simulink model "LOS_Tracking"  (R2021b)
settings: Solver=VariableStepAuto  StartTime=0.0  StopTime=273.72  RelTol=1e-3
values from neighbouring files (symbols this model uses):
  EL = out.EL    [plot_result.m]
undefined symbols (not defined in the file or in its folder): AZ, Optics
libraries: slpidlib x10, simulink_extras x10
(part 1 of 2)
settings Model: Creator=NGOC MAI  LastModifiedBy=NGOC MAI
settings DebuggingCC: UnconnectedInputMsg=none  UnconnectedOutputMsg=none  UnconnectedLineMsg=none
settings ModelReferenceCC: EnableRefExpFcnMdlSchedulingChecks=off
settings RTWCC: DLArmComputeVersion=20.02.1

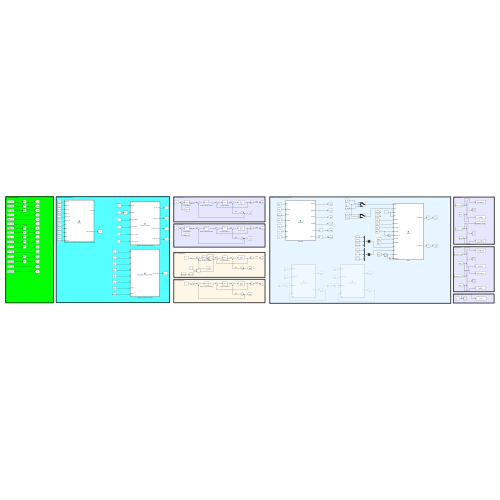
[thumbnail: Simulink's stored preview of the top-level diagram]
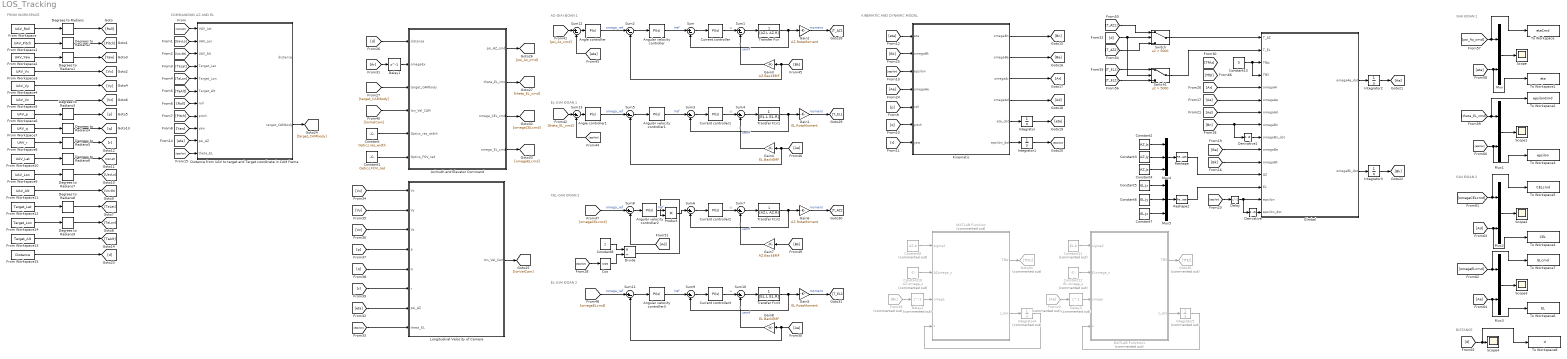
== system LOS_Tracking ==
  note: DISTANCE
  note: GIAI ĐOẠN 2
  note: GIAI ĐOẠN 1
  note: COMMANDING AZ AND EL
  note: FROM WORKSPACE
  note: KINEMATIC AND DYNAMIC MODEL
  note: AZ-GIAI ĐOẠN 1
  note: EL-GIAI ĐOẠN 1
  note: EL-GIAI ĐOẠN 2
  note: CEL-GIAI ĐOẠN 2
  Angle controller : slpidlib/PID Controller  Controller=P  Form=Parallel  TimeDomain=Continuous-time  UseExternalTs=off  SampleTime=-1  IntegratorMethod=Forward Euler  FilterMethod=Forward Euler  ControllerParametersSource=internal  P=AZ.KPpos  I=1  D=0  N=100  UseFilter=on  TunerSelectOption=Transfer Function Based (PID Tuner App)  InitialConditionSource=internal  InitialConditionForIntegrator=0  InitialConditionForFilter=0  DifferentiatorICPrevScaledInput=0  ExternalReset=none  TrackingMode=off  Kt=1  LimitOutput=off  SatLimitsSource=internal  UpperSaturationLimit=inf  LowerSaturationLimit=-inf  LinearizeAsGain=on  AntiWindupMode=none  Kb=1  POutMin=[]  POutMax=[]  IOutMin=[]  IOutMax=[]  DOutMin=[]  DOutMax=[]  NOutMin=[]  NOutMax=[]  SumOutMin=[]  SumOutMax=[]  SaturationOutMin=[]  SaturationOutMax=[]  PParamMin=[]  PParamMax=[]  IParamMin=[]  IParamMax=[]  DParamMin=[]  DParamMax=[]  NParamMin=[]  NParamMax=[]  KbParamMin=[]  KbParamMax=[]  KtParamMin=[]  KtParamMax=[]  KbOutMin=[]  KbOutMax=[]  KtOutMin=[]  KtOutMax=[]  IntegratorOutMin=[]  IntegratorOutMax=[]  FilterOutMin=[]  FilterOutMax=[]  SumI1OutMin=[]  SumI1OutMax=[]  SumI2OutMin=[]  SumI2OutMax=[]  SumI3OutMin=[]  SumI3OutMax=[]  SumI4OutMin=[]  SumI4OutMax=[]  SumDOutMin=[]  SumDOutMax=[]  DifferentiatorOutMin=[]  DifferentiatorOutMax=[]  FilterDiffOutCoefMin=[]  FilterDiffOutCoefMax=[]  ReciprocalOutMin=[]  ReciprocalOutMax=[]  SumDenOutMin=[]  SumDenOutMax=[]  SumNumOutMin=[]  SumNumOutMax=[]  DivideOutMin=[]  DivideOutMax=[]  UdiffTsProdOutMin=[]  UdiffTsProdOutMax=[]  NTsProdOutMin=[]  NTsProdOutMax=[]  UintegralTsProdOutMin=[]  UintegralTsProdOutMax=[]  UngainTsProdOutMin=[]  UngainTsProdOutMax=[]  IntegratorContinuousStateAttributes=''  IntegratorStateMustResolveToSignalObject=off  IntegratorRTWStateStorageClass=Auto  FilterContinuousStateAttributes=''  FilterStateMustResolveToSignalObject=off  FilterRTWStateStorageClass=Auto  ParallelPVariant=InternalParameters  IdealPVariant=Disabled  IVariant=Disabled  DVariant=Disabled  IntegratorVariant=Disabled  SatVariant=Disabled  AWVariant=Disabled  PCopyVariant=Disabled  TRVariant=Disabled  FdbkBlocksVariant=Forward  IdealPFdbkVariant=Disabled  SatFdbkVariant=Disabled  DerivativeFilterVariant=Disabled  NVariant=Disabled  NCopyVariant=Disabled_SignalSpec  FilterICVariant=Disabled  IntegratorICVariant=Disabled  ExternalResetVariant=Disabled  TRSumVariant=Passthrough  SumFdbkVariant=Disabled  SumVariant=Passthrough_P  TsampFilterVariant=InternalTs  TsampNgainVariant=Passthrough  TsampIntegralVariant=Disabled_SignalSpec  ExternalSaturationOutDataTypeStr=Inherit: Same as second input
  Angle controller1 : slpidlib/PID Controller  Controller=P  Form=Parallel  TimeDomain=Continuous-time  UseExternalTs=off  SampleTime=-1  IntegratorMethod=Forward Euler  FilterMethod=Forward Euler  ControllerParametersSource=internal  P=EL.KPpos  I=1  D=0  N=100  UseFilter=on  TunerSelectOption=Transfer Function Based (PID Tuner App)  InitialConditionSource=internal  InitialConditionForIntegrator=0  InitialConditionForFilter=0  DifferentiatorICPrevScaledInput=0  ExternalReset=none  TrackingMode=off  Kt=1  LimitOutput=off  SatLimitsSource=internal  UpperSaturationLimit=inf  LowerSaturationLimit=-inf  LinearizeAsGain=on  AntiWindupMode=none  Kb=1  POutMin=[]  POutMax=[]  IOutMin=[]  IOutMax=[]  DOutMin=[]  DOutMax=[]  NOutMin=[]  NOutMax=[]  SumOutMin=[]  SumOutMax=[]  SaturationOutMin=[]  SaturationOutMax=[]  PParamMin=[]  PParamMax=[]  IParamMin=[]  IParamMax=[]  DParamMin=[]  DParamMax=[]  NParamMin=[]  NParamMax=[]  KbParamMin=[]  KbParamMax=[]  KtParamMin=[]  KtParamMax=[]  KbOutMin=[]  KbOutMax=[]  KtOutMin=[]  KtOutMax=[]  IntegratorOutMin=[]  IntegratorOutMax=[]  FilterOutMin=[]  FilterOutMax=[]  SumI1OutMin=[]  SumI1OutMax=[]  SumI2OutMin=[]  SumI2OutMax=[]  SumI3OutMin=[]  SumI3OutMax=[]  SumI4OutMin=[]  SumI4OutMax=[]  SumDOutMin=[]  SumDOutMax=[]  DifferentiatorOutMin=[]  DifferentiatorOutMax=[]  FilterDiffOutCoefMin=[]  FilterDiffOutCoefMax=[]  ReciprocalOutMin=[]  ReciprocalOutMax=[]  SumDenOutMin=[]  SumDenOutMax=[]  SumNumOutMin=[]  SumNumOutMax=[]  DivideOutMin=[]  DivideOutMax=[]  UdiffTsProdOutMin=[]  UdiffTsProdOutMax=[]  NTsProdOutMin=[]  NTsProdOutMax=[]  UintegralTsProdOutMin=[]  UintegralTsProdOutMax=[]  UngainTsProdOutMin=[]  UngainTsProdOutMax=[]  IntegratorContinuousStateAttributes=''  IntegratorStateMustResolveToSignalObject=off  IntegratorRTWStateStorageClass=Auto  FilterContinuousStateAttributes=''  FilterStateMustResolveToSignalObject=off  FilterRTWStateStorageClass=Auto  ParallelPVariant=InternalParameters  IdealPVariant=Disabled  IVariant=Disabled  DVariant=Disabled  IntegratorVariant=Disabled  SatVariant=Disabled  AWVariant=Disabled  PCopyVariant=Disabled  TRVariant=Disabled  FdbkBlocksVariant=Forward  IdealPFdbkVariant=Disabled  SatFdbkVariant=Disabled  DerivativeFilterVariant=Disabled  NVariant=Disabled  NCopyVariant=Disabled_SignalSpec  FilterICVariant=Disabled  IntegratorICVariant=Disabled  ExternalResetVariant=Disabled  TRSumVariant=Passthrough  SumFdbkVariant=Disabled  SumVariant=Passthrough_P  TsampFilterVariant=InternalTs  TsampNgainVariant=Passthrough  TsampIntegralVariant=Disabled_SignalSpec  ExternalSaturationOutDataTypeStr=Inherit: Same as second input
  Angular velocity controller : slpidlib/PID Controller  Controller=PI  Form=Parallel  TimeDomain=Continuous-time  UseExternalTs=off  SampleTime=-1  IntegratorMethod=Forward Euler  FilterMethod=Forward Euler  ControllerParametersSource=internal  P=AZ.KPvel  I=AZ.KIvel  D=0  N=100  UseFilter=on  TunerSelectOption=Transfer Function Based (PID Tuner App)  InitialConditionSource=internal  InitialConditionForIntegrator=0  InitialConditionForFilter=0  DifferentiatorICPrevScaledInput=0  ExternalReset=none  TrackingMode=off  Kt=1  LimitOutput=off  SatLimitsSource=internal  UpperSaturationLimit=inf  LowerSaturationLimit=-inf  LinearizeAsGain=on  AntiWindupMode=none  Kb=1  POutMin=[]  POutMax=[]  IOutMin=[]  IOutMax=[]  DOutMin=[]  DOutMax=[]  NOutMin=[]  NOutMax=[]  SumOutMin=[]  SumOutMax=[]  SaturationOutMin=[]  SaturationOutMax=[]  PParamMin=[]  PParamMax=[]  IParamMin=[]  IParamMax=[]  DParamMin=[]  DParamMax=[]  NParamMin=[]  NParamMax=[]  KbParamMin=[]  KbParamMax=[]  KtParamMin=[]  KtParamMax=[]  KbOutMin=[]  KbOutMax=[]  KtOutMin=[]  KtOutMax=[]  IntegratorOutMin=[]  IntegratorOutMax=[]  FilterOutMin=[]  FilterOutMax=[]  SumI1OutMin=[]  SumI1OutMax=[]  SumI2OutMin=[]  SumI2OutMax=[]  SumI3OutMin=[]  SumI3OutMax=[]  SumI4OutMin=[]  SumI4OutMax=[]  SumDOutMin=[]  SumDOutMax=[]  DifferentiatorOutMin=[]  DifferentiatorOutMax=[]  FilterDiffOutCoefMin=[]  FilterDiffOutCoefMax=[]  ReciprocalOutMin=[]  ReciprocalOutMax=[]  SumDenOutMin=[]  SumDenOutMax=[]  SumNumOutMin=[]  SumNumOutMax=[]  DivideOutMin=[]  DivideOutMax=[]  UdiffTsProdOutMin=[]  UdiffTsProdOutMax=[]  NTsProdOutMin=[]  NTsProdOutMax=[]  UintegralTsProdOutMin=[]  UintegralTsProdOutMax=[]  UngainTsProdOutMin=[]  UngainTsProdOutMax=[]  IntegratorContinuousStateAttributes=''  IntegratorStateMustResolveToSignalObject=off  IntegratorRTWStateStorageClass=Auto  FilterContinuousStateAttributes=''  FilterStateMustResolveToSignalObject=off  FilterRTWStateStorageClass=Auto  ParallelPVariant=InternalParameters  IdealPVariant=Disabled  IVariant=InternalParameters  DVariant=Disabled  IntegratorVariant=Continuous  SatVariant=Disabled  AWVariant=Passthrough  PCopyVariant=Disabled  TRVariant=Disabled  FdbkBlocksVariant=Forward  IdealPFdbkVariant=Disabled  SatFdbkVariant=Disabled  DerivativeFilterVariant=Disabled  NVariant=Disabled  NCopyVariant=Disabled_SignalSpec  FilterICVariant=Disabled  IntegratorICVariant=InternalICs  ExternalResetVariant=Disabled  TRSumVariant=Passthrough  SumFdbkVariant=Disabled  SumVariant=Sum_PI  TsampFilterVariant=InternalTs  TsampNgainVariant=Passthrough  TsampIntegralVariant=Disabled_SignalSpec  ExternalSaturationOutDataTypeStr=Inherit: Same as second input
  Angular velocity controller1 : slpidlib/PID Controller  Controller=PI  Form=Parallel  TimeDomain=Continuous-time  UseExternalTs=off  SampleTime=-1  IntegratorMethod=Forward Euler  FilterMethod=Forward Euler  ControllerParametersSource=internal  P=EL.KPvel  I=EL.KIvel  D=0  N=100  UseFilter=on  TunerSelectOption=Transfer Function Based (PID Tuner App)  InitialConditionSource=internal  InitialConditionForIntegrator=0  InitialConditionForFilter=0  DifferentiatorICPrevScaledInput=0  ExternalReset=none  TrackingMode=off  Kt=1  LimitOutput=off  SatLimitsSource=internal  UpperSaturationLimit=inf  LowerSaturationLimit=-inf  LinearizeAsGain=on  AntiWindupMode=none  Kb=1  POutMin=[]  POutMax=[]  IOutMin=[]  IOutMax=[]  DOutMin=[]  DOutMax=[]  NOutMin=[]  NOutMax=[]  SumOutMin=[]  SumOutMax=[]  SaturationOutMin=[]  SaturationOutMax=[]  PParamMin=[]  PParamMax=[]  IParamMin=[]  IParamMax=[]  DParamMin=[]  DParamMax=[]  NParamMin=[]  NParamMax=[]  KbParamMin=[]  KbParamMax=[]  KtParamMin=[]  KtParamMax=[]  KbOutMin=[]  KbOutMax=[]  KtOutMin=[]  KtOutMax=[]  IntegratorOutMin=[]  IntegratorOutMax=[]  FilterOutMin=[]  FilterOutMax=[]  SumI1OutMin=[]  SumI1OutMax=[]  SumI2OutMin=[]  SumI2OutMax=[]  SumI3OutMin=[]  SumI3OutMax=[]  SumI4OutMin=[]  SumI4OutMax=[]  SumDOutMin=[]  SumDOutMax=[]  DifferentiatorOutMin=[]  DifferentiatorOutMax=[]  FilterDiffOutCoefMin=[]  FilterDiffOutCoefMax=[]  ReciprocalOutMin=[]  ReciprocalOutMax=[]  SumDenOutMin=[]  SumDenOutMax=[]  SumNumOutMin=[]  SumNumOutMax=[]  DivideOutMin=[]  DivideOutMax=[]  UdiffTsProdOutMin=[]  UdiffTsProdOutMax=[]  NTsProdOutMin=[]  NTsProdOutMax=[]  UintegralTsProdOutMin=[]  UintegralTsProdOutMax=[]  UngainTsProdOutMin=[]  UngainTsProdOutMax=[]  IntegratorContinuousStateAttributes=''  IntegratorStateMustResolveToSignalObject=off  IntegratorRTWStateStorageClass=Auto  FilterContinuousStateAttributes=''  FilterStateMustResolveToSignalObject=off  FilterRTWStateStorageClass=Auto  ParallelPVariant=InternalParameters  IdealPVariant=Disabled  IVariant=InternalParameters  DVariant=Disabled  IntegratorVariant=Continuous  SatVariant=Disabled  AWVariant=Passthrough  PCopyVariant=Disabled  TRVariant=Disabled  FdbkBlocksVariant=Forward  IdealPFdbkVariant=Disabled  SatFdbkVariant=Disabled  DerivativeFilterVariant=Disabled  NVariant=Disabled  NCopyVariant=Disabled_SignalSpec  FilterICVariant=Disabled  IntegratorICVariant=InternalICs  ExternalResetVariant=Disabled  TRSumVariant=Passthrough  SumFdbkVariant=Disabled  SumVariant=Sum_PI  TsampFilterVariant=InternalTs  TsampNgainVariant=Passthrough  TsampIntegralVariant=Disabled_SignalSpec  ExternalSaturationOutDataTypeStr=Inherit: Same as second input
  Angular velocity controller2 : slpidlib/PID Controller  Controller=PI  Form=Parallel  TimeDomain=Continuous-time  UseExternalTs=off  SampleTime=-1  IntegratorMethod=Forward Euler  FilterMethod=Forward Euler  ControllerParametersSource=internal  P=AZ.KPvel  I=AZ.KIvel  D=0  N=100  UseFilter=on  TunerSelectOption=Transfer Function Based (PID Tuner App)  InitialConditionSource=internal  InitialConditionForIntegrator=0  InitialConditionForFilter=0  DifferentiatorICPrevScaledInput=0  ExternalReset=none  TrackingMode=off  Kt=1  LimitOutput=off  SatLimitsSource=internal  UpperSaturationLimit=inf  LowerSaturationLimit=-inf  LinearizeAsGain=on  AntiWindupMode=none  Kb=1  POutMin=[]  POutMax=[]  IOutMin=[]  IOutMax=[]  DOutMin=[]  DOutMax=[]  NOutMin=[]  NOutMax=[]  SumOutMin=[]  SumOutMax=[]  SaturationOutMin=[]  SaturationOutMax=[]  PParamMin=[]  PParamMax=[]  IParamMin=[]  IParamMax=[]  DParamMin=[]  DParamMax=[]  NParamMin=[]  NParamMax=[]  KbParamMin=[]  KbParamMax=[]  KtParamMin=[]  KtParamMax=[]  KbOutMin=[]  KbOutMax=[]  KtOutMin=[]  KtOutMax=[]  IntegratorOutMin=[]  IntegratorOutMax=[]  FilterOutMin=[]  FilterOutMax=[]  SumI1OutMin=[]  SumI1OutMax=[]  SumI2OutMin=[]  SumI2OutMax=[]  SumI3OutMin=[]  SumI3OutMax=[]  SumI4OutMin=[]  SumI4OutMax=[]  SumDOutMin=[]  SumDOutMax=[]  DifferentiatorOutMin=[]  DifferentiatorOutMax=[]  FilterDiffOutCoefMin=[]  FilterDiffOutCoefMax=[]  ReciprocalOutMin=[]  ReciprocalOutMax=[]  SumDenOutMin=[]  SumDenOutMax=[]  SumNumOutMin=[]  SumNumOutMax=[]  DivideOutMin=[]  DivideOutMax=[]  UdiffTsProdOutMin=[]  UdiffTsProdOutMax=[]  NTsProdOutMin=[]  NTsProdOutMax=[]  UintegralTsProdOutMin=[]  UintegralTsProdOutMax=[]  UngainTsProdOutMin=[]  UngainTsProdOutMax=[]  IntegratorContinuousStateAttributes=''  IntegratorStateMustResolveToSignalObject=off  IntegratorRTWStateStorageClass=Auto  FilterContinuousStateAttributes=''  FilterStateMustResolveToSignalObject=off  FilterRTWStateStorageClass=Auto  ParallelPVariant=InternalParameters  IdealPVariant=Disabled  IVariant=InternalParameters  DVariant=Disabled  IntegratorVariant=Continuous  SatVariant=Disabled  AWVariant=Passthrough  PCopyVariant=Disabled  TRVariant=Disabled  FdbkBlocksVariant=Forward  IdealPFdbkVariant=Disabled  SatFdbkVariant=Disabled  DerivativeFilterVariant=Disabled  NVariant=Disabled  NCopyVariant=Disabled_SignalSpec  FilterICVariant=Disabled  IntegratorICVariant=InternalICs  ExternalResetVariant=Disabled  TRSumVariant=Passthrough  SumFdbkVariant=Disabled  SumVariant=Sum_PI  TsampFilterVariant=InternalTs  TsampNgainVariant=Passthrough  TsampIntegralVariant=Disabled_SignalSpec  ExternalSaturationOutDataTypeStr=Inherit: Same as second input
  Angular velocity controller3 : slpidlib/PID Controller  Controller=PI  Form=Parallel  TimeDomain=Continuous-time  UseExternalTs=off  SampleTime=-1  IntegratorMethod=Forward Euler  FilterMethod=Forward Euler  ControllerParametersSource=internal  P=EL.KPvel  I=EL.KIvel  D=0  N=100  UseFilter=on  TunerSelectOption=Transfer Function Based (PID Tuner App)  InitialConditionSource=internal  InitialConditionForIntegrator=0  InitialConditionForFilter=0  DifferentiatorICPrevScaledInput=0  ExternalReset=none  TrackingMode=off  Kt=1  LimitOutput=off  SatLimitsSource=internal  UpperSaturationLimit=inf  LowerSaturationLimit=-inf  LinearizeAsGain=on  AntiWindupMode=none  Kb=1  POutMin=[]  POutMax=[]  IOutMin=[]  IOutMax=[]  DOutMin=[]  DOutMax=[]  NOutMin=[]  NOutMax=[]  SumOutMin=[]  SumOutMax=[]  SaturationOutMin=[]  SaturationOutMax=[]  PParamMin=[]  PParamMax=[]  IParamMin=[]  IParamMax=[]  DParamMin=[]  DParamMax=[]  NParamMin=[]  NParamMax=[]  KbParamMin=[]  KbParamMax=[]  KtParamMin=[]  KtParamMax=[]  KbOutMin=[]  KbOutMax=[]  KtOutMin=[]  KtOutMax=[]  IntegratorOutMin=[]  IntegratorOutMax=[]  FilterOutMin=[]  FilterOutMax=[]  SumI1OutMin=[]  SumI1OutMax=[]  SumI2OutMin=[]  SumI2OutMax=[]  SumI3OutMin=[]  SumI3OutMax=[]  SumI4OutMin=[]  SumI4OutMax=[]  SumDOutMin=[]  SumDOutMax=[]  DifferentiatorOutMin=[]  DifferentiatorOutMax=[]  FilterDiffOutCoefMin=[]  FilterDiffOutCoefMax=[]  ReciprocalOutMin=[]  ReciprocalOutMax=[]  SumDenOutMin=[]  SumDenOutMax=[]  SumNumOutMin=[]  SumNumOutMax=[]  DivideOutMin=[]  DivideOutMax=[]  UdiffTsProdOutMin=[]  UdiffTsProdOutMax=[]  NTsProdOutMin=[]  NTsProdOutMax=[]  UintegralTsProdOutMin=[]  UintegralTsProdOutMax=[]  UngainTsProdOutMin=[]  UngainTsProdOutMax=[]  IntegratorContinuousStateAttributes=''  IntegratorStateMustResolveToSignalObject=off  IntegratorRTWStateStorageClass=Auto  FilterContinuousStateAttributes=''  FilterStateMustResolveToSignalObject=off  FilterRTWStateStorageClass=Auto  ParallelPVariant=InternalParameters  IdealPVariant=Disabled  IVariant=InternalParameters  DVariant=Disabled  IntegratorVariant=Continuous  SatVariant=Disabled  AWVariant=Passthrough  PCopyVariant=Disabled  TRVariant=Disabled  FdbkBlocksVariant=Forward  IdealPFdbkVariant=Disabled  SatFdbkVariant=Disabled  DerivativeFilterVariant=Disabled  NVariant=Disabled  NCopyVariant=Disabled_SignalSpec  FilterICVariant=Disabled  IntegratorICVariant=InternalICs  ExternalResetVariant=Disabled  TRSumVariant=Passthrough  SumFdbkVariant=Disabled  SumVariant=Sum_PI  TsampFilterVariant=InternalTs  TsampNgainVariant=Passthrough  TsampIntegralVariant=Disabled_SignalSpec  ExternalSaturationOutDataTypeStr=Inherit: Same as second input
  Azimuth and Elevator Command : MATLAB Function  TreatAsAtomicUnit=on
  Constant : Constant  Value=Optics.res_width
  Constant1 : Constant  Value=Optics.FOV_rad
  Constant10 : Constant  Commented=on  Value=AZ.omega_s
  Constant11 : Constant  Commented=on  Value=EL.b
  Constant12 : Constant  Commented=on  Value=EL.omega_s
  Constant13 : Constant  Value=0
  Constant2 : Constant  Value=AZ.Jx
  Constant3 : Constant  Value=AZ.Jy
  Constant4 : Constant  Value=AZ.Jz
  Constant5 : Constant  Value=EL.Jx
  Constant6 : Constant  Value=EL.Jy
  Constant7 : Constant  Value=EL.Jz
  Constant8 : Constant
  Constant9 : Constant  Commented=on  Value=AZ.b
  Cos : Trigonometry  Operator=cos
  Current controller : slpidlib/PID Controller  Controller=PI  Form=Parallel  TimeDomain=Continuous-time  UseExternalTs=off  SampleTime=-1  IntegratorMethod=Forward Euler  FilterMethod=Forward Euler  ControllerParametersSource=internal  P=AZ.KPcurrent  I=AZ.KIcurrent  D=0  N=100  UseFilter=on  TunerSelectOption=Transfer Function Based (PID Tuner App)  InitialConditionSource=internal  InitialConditionForIntegrator=0  InitialConditionForFilter=0  DifferentiatorICPrevScaledInput=0  ExternalReset=none  TrackingMode=off  Kt=1  LimitOutput=off  SatLimitsSource=internal  UpperSaturationLimit=inf  LowerSaturationLimit=-inf  LinearizeAsGain=on  AntiWindupMode=none  Kb=1  POutMin=[]  POutMax=[]  IOutMin=[]  IOutMax=[]  DOutMin=[]  DOutMax=[]  NOutMin=[]  NOutMax=[]  SumOutMin=[]  SumOutMax=[]  SaturationOutMin=[]  SaturationOutMax=[]  PParamMin=[]  PParamMax=[]  IParamMin=[]  IParamMax=[]  DParamMin=[]  DParamMax=[]  NParamMin=[]  NParamMax=[]  KbParamMin=[]  KbParamMax=[]  KtParamMin=[]  KtParamMax=[]  KbOutMin=[]  KbOutMax=[]  KtOutMin=[]  KtOutMax=[]  IntegratorOutMin=[]  IntegratorOutMax=[]  FilterOutMin=[]  FilterOutMax=[]  SumI1OutMin=[]  SumI1OutMax=[]  SumI2OutMin=[]  SumI2OutMax=[]  SumI3OutMin=[]  SumI3OutMax=[]  SumI4OutMin=[]  SumI4OutMax=[]  SumDOutMin=[]  SumDOutMax=[]  DifferentiatorOutMin=[]  DifferentiatorOutMax=[]  FilterDiffOutCoefMin=[]  FilterDiffOutCoefMax=[]  ReciprocalOutMin=[]  ReciprocalOutMax=[]  SumDenOutMin=[]  SumDenOutMax=[]  SumNumOutMin=[]  SumNumOutMax=[]  DivideOutMin=[]  DivideOutMax=[]  UdiffTsProdOutMin=[]  UdiffTsProdOutMax=[]  NTsProdOutMin=[]  NTsProdOutMax=[]  UintegralTsProdOutMin=[]  UintegralTsProdOutMax=[]  UngainTsProdOutMin=[]  UngainTsProdOutMax=[]  IntegratorContinuousStateAttributes=''  IntegratorStateMustResolveToSignalObject=off  IntegratorRTWStateStorageClass=Auto  FilterContinuousStateAttributes=''  FilterStateMustResolveToSignalObject=off  FilterRTWStateStorageClass=Auto  ParallelPVariant=InternalParameters  IdealPVariant=Disabled  IVariant=InternalParameters  DVariant=Disabled  IntegratorVariant=Continuous  SatVariant=Disabled  AWVariant=Passthrough  PCopyVariant=Disabled  TRVariant=Disabled  FdbkBlocksVariant=Forward  IdealPFdbkVariant=Disabled  SatFdbkVariant=Disabled  DerivativeFilterVariant=Disabled  NVariant=Disabled  NCopyVariant=Disabled_SignalSpec  FilterICVariant=Disabled  IntegratorICVariant=InternalICs  ExternalResetVariant=Disabled  TRSumVariant=Passthrough  SumFdbkVariant=Disabled  SumVariant=Sum_PI  TsampFilterVariant=InternalTs  TsampNgainVariant=Passthrough  TsampIntegralVariant=Disabled_SignalSpec  ExternalSaturationOutDataTypeStr=Inherit: Same as second input
  Current controller1 : slpidlib/PID Controller  Controller=PI  Form=Parallel  TimeDomain=Continuous-time  UseExternalTs=off  SampleTime=-1  IntegratorMethod=Forward Euler  FilterMethod=Forward Euler  ControllerParametersSource=internal  P=EL.KPcurrent  I=EL.KIcurrent  D=0  N=100  UseFilter=on  TunerSelectOption=Transfer Function Based (PID Tuner App)  InitialConditionSource=internal  InitialConditionForIntegrator=0  InitialConditionForFilter=0  DifferentiatorICPrevScaledInput=0  ExternalReset=none  TrackingMode=off  Kt=1  LimitOutput=off  SatLimitsSource=internal  UpperSaturationLimit=inf  LowerSaturationLimit=-inf  LinearizeAsGain=on  AntiWindupMode=none  Kb=1  POutMin=[]  POutMax=[]  IOutMin=[]  IOutMax=[]  DOutMin=[]  DOutMax=[]  NOutMin=[]  NOutMax=[]  SumOutMin=[]  SumOutMax=[]  SaturationOutMin=[]  SaturationOutMax=[]  PParamMin=[]  PParamMax=[]  IParamMin=[]  IParamMax=[]  DParamMin=[]  DParamMax=[]  NParamMin=[]  NParamMax=[]  KbParamMin=[]  KbParamMax=[]  KtParamMin=[]  KtParamMax=[]  KbOutMin=[]  KbOutMax=[]  KtOutMin=[]  KtOutMax=[]  IntegratorOutMin=[]  IntegratorOutMax=[]  FilterOutMin=[]  FilterOutMax=[]  SumI1OutMin=[]  SumI1OutMax=[]  SumI2OutMin=[]  SumI2OutMax=[]  SumI3OutMin=[]  SumI3OutMax=[]  SumI4OutMin=[]  SumI4OutMax=[]  SumDOutMin=[]  SumDOutMax=[]  DifferentiatorOutMin=[]  DifferentiatorOutMax=[]  FilterDiffOutCoefMin=[]  FilterDiffOutCoefMax=[]  ReciprocalOutMin=[]  ReciprocalOutMax=[]  SumDenOutMin=[]  SumDenOutMax=[]  SumNumOutMin=[]  SumNumOutMax=[]  DivideOutMin=[]  DivideOutMax=[]  UdiffTsProdOutMin=[]  UdiffTsProdOutMax=[]  NTsProdOutMin=[]  NTsProdOutMax=[]  UintegralTsProdOutMin=[]  UintegralTsProdOutMax=[]  UngainTsProdOutMin=[]  UngainTsProdOutMax=[]  IntegratorContinuousStateAttributes=''  IntegratorStateMustResolveToSignalObject=off  IntegratorRTWStateStorageClass=Auto  FilterContinuousStateAttributes=''  FilterStateMustResolveToSignalObject=off  FilterRTWStateStorageClass=Auto  ParallelPVariant=InternalParameters  IdealPVariant=Disabled  IVariant=InternalParameters  DVariant=Disabled  IntegratorVariant=Continuous  SatVariant=Disabled  AWVariant=Passthrough  PCopyVariant=Disabled  TRVariant=Disabled  FdbkBlocksVariant=Forward  IdealPFdbkVariant=Disabled  SatFdbkVariant=Disabled  DerivativeFilterVariant=Disabled  NVariant=Disabled  NCopyVariant=Disabled_SignalSpec  FilterICVariant=Disabled  IntegratorICVariant=InternalICs  ExternalResetVariant=Disabled  TRSumVariant=Passthrough  SumFdbkVariant=Disabled  SumVariant=Sum_PI  TsampFilterVariant=InternalTs  TsampNgainVariant=Passthrough  TsampIntegralVariant=Disabled_SignalSpec  ExternalSaturationOutDataTypeStr=Inherit: Same as second input
  Current controller2 : slpidlib/PID Controller  Controller=PI  Form=Parallel  TimeDomain=Continuous-time  UseExternalTs=off  SampleTime=-1  IntegratorMethod=Forward Euler  FilterMethod=Forward Euler  ControllerParametersSource=internal  P=AZ.KPcurrent  I=AZ.KIcurrent  D=0  N=100  UseFilter=on  TunerSelectOption=Transfer Function Based (PID Tuner App)  InitialConditionSource=internal  InitialConditionForIntegrator=0  InitialConditionForFilter=0  DifferentiatorICPrevScaledInput=0  ExternalReset=none  TrackingMode=off  Kt=1  LimitOutput=off  SatLimitsSource=internal  UpperSaturationLimit=inf  LowerSaturationLimit=-inf  LinearizeAsGain=on  AntiWindupMode=none  Kb=1  POutMin=[]  POutMax=[]  IOutMin=[]  IOutMax=[]  DOutMin=[]  DOutMax=[]  NOutMin=[]  NOutMax=[]  SumOutMin=[]  SumOutMax=[]  SaturationOutMin=[]  SaturationOutMax=[]  PParamMin=[]  PParamMax=[]  IParamMin=[]  IParamMax=[]  DParamMin=[]  DParamMax=[]  NParamMin=[]  NParamMax=[]  KbParamMin=[]  KbParamMax=[]  KtParamMin=[]  KtParamMax=[]  KbOutMin=[]  KbOutMax=[]  KtOutMin=[]  KtOutMax=[]  IntegratorOutMin=[]  IntegratorOutMax=[]  FilterOutMin=[]  FilterOutMax=[]  SumI1OutMin=[]  SumI1OutMax=[]  SumI2OutMin=[]  SumI2OutMax=[]  SumI3OutMin=[]  SumI3OutMax=[]  SumI4OutMin=[]  SumI4OutMax=[]  SumDOutMin=[]  SumDOutMax=[]  DifferentiatorOutMin=[]  DifferentiatorOutMax=[]  FilterDiffOutCoefMin=[]  FilterDiffOutCoefMax=[]  ReciprocalOutMin=[]  ReciprocalOutMax=[]  SumDenOutMin=[]  SumDenOutMax=[]  SumNumOutMin=[]  SumNumOutMax=[]  DivideOutMin=[]  DivideOutMax=[]  UdiffTsProdOutMin=[]  UdiffTsProdOutMax=[]  NTsProdOutMin=[]  NTsProdOutMax=[]  UintegralTsProdOutMin=[]  UintegralTsProdOutMax=[]  UngainTsProdOutMin=[]  UngainTsProdOutMax=[]  IntegratorContinuousStateAttributes=''  IntegratorStateMustResolveToSignalObject=off  IntegratorRTWStateStorageClass=Auto  FilterContinuousStateAttributes=''  FilterStateMustResolveToSignalObject=off  FilterRTWStateStorageClass=Auto  ParallelPVariant=InternalParameters  IdealPVariant=Disabled  IVariant=InternalParameters  DVariant=Disabled  IntegratorVariant=Continuous  SatVariant=Disabled  AWVariant=Passthrough  PCopyVariant=Disabled  TRVariant=Disabled  FdbkBlocksVariant=Forward  IdealPFdbkVariant=Disabled  SatFdbkVariant=Disabled  DerivativeFilterVariant=Disabled  NVariant=Disabled  NCopyVariant=Disabled_SignalSpec  FilterICVariant=Disabled  IntegratorICVariant=InternalICs  ExternalResetVariant=Disabled  TRSumVariant=Passthrough  SumFdbkVariant=Disabled  SumVariant=Sum_PI  TsampFilterVariant=InternalTs  TsampNgainVariant=Passthrough  TsampIntegralVariant=Disabled_SignalSpec  ExternalSaturationOutDataTypeStr=Inherit: Same as second input
  Current controller3 : slpidlib/PID Controller  Controller=PI  Form=Parallel  TimeDomain=Continuous-time  UseExternalTs=off  SampleTime=-1  IntegratorMethod=Forward Euler  FilterMethod=Forward Euler  ControllerParametersSource=internal  P=EL.KPcurrent  I=EL.KIcurrent  D=0  N=100  UseFilter=on  TunerSelectOption=Transfer Function Based (PID Tuner App)  InitialConditionSource=internal  InitialConditionForIntegrator=0  InitialConditionForFilter=0  DifferentiatorICPrevScaledInput=0  ExternalReset=none  TrackingMode=off  Kt=1  LimitOutput=off  SatLimitsSource=internal  UpperSaturationLimit=inf  LowerSaturationLimit=-inf  LinearizeAsGain=on  AntiWindupMode=none  Kb=1  POutMin=[]  POutMax=[]  IOutMin=[]  IOutMax=[]  DOutMin=[]  DOutMax=[]  NOutMin=[]  NOutMax=[]  SumOutMin=[]  SumOutMax=[]  SaturationOutMin=[]  SaturationOutMax=[]  PParamMin=[]  PParamMax=[]  IParamMin=[]  IParamMax=[]  DParamMin=[]  DParamMax=[]  NParamMin=[]  NParamMax=[]  KbParamMin=[]  KbParamMax=[]  KtParamMin=[]  KtParamMax=[]  KbOutMin=[]  KbOutMax=[]  KtOutMin=[]  KtOutMax=[]  IntegratorOutMin=[]  IntegratorOutMax=[]  FilterOutMin=[]  FilterOutMax=[]  SumI1OutMin=[]  SumI1OutMax=[]  SumI2OutMin=[]  SumI2OutMax=[]  SumI3OutMin=[]  SumI3OutMax=[]  SumI4OutMin=[]  SumI4OutMax=[]  SumDOutMin=[]  SumDOutMax=[]  DifferentiatorOutMin=[]  DifferentiatorOutMax=[]  FilterDiffOutCoefMin=[]  FilterDiffOutCoefMax=[]  ReciprocalOutMin=[]  ReciprocalOutMax=[]  SumDenOutMin=[]  SumDenOutMax=[]  SumNumOutMin=[]  SumNumOutMax=[]  DivideOutMin=[]  DivideOutMax=[]  UdiffTsProdOutMin=[]  UdiffTsProdOutMax=[]  NTsProdOutMin=[]  NTsProdOutMax=[]  UintegralTsProdOutMin=[]  UintegralTsProdOutMax=[]  UngainTsProdOutMin=[]  UngainTsProdOutMax=[]  IntegratorContinuousStateAttributes=''  IntegratorStateMustResolveToSignalObject=off  IntegratorRTWStateStorageClass=Auto  FilterContinuousStateAttributes=''  FilterStateMustResolveToSignalObject=off  FilterRTWStateStorageClass=Auto  ParallelPVariant=InternalParameters  IdealPVariant=Disabled  IVariant=InternalParameters  DVariant=Disabled  IntegratorVariant=Continuous  SatVariant=Disabled  AWVariant=Passthrough  PCopyVariant=Disabled  TRVariant=Disabled  FdbkBlocksVariant=Forward  IdealPFdbkVariant=Disabled  SatFdbkVariant=Disabled  DerivativeFilterVariant=Disabled  NVariant=Disabled  NCopyVariant=Disabled_SignalSpec  FilterICVariant=Disabled  IntegratorICVariant=InternalICs  ExternalResetVariant=Disabled  TRSumVariant=Passthrough  SumFdbkVariant=Disabled  SumVariant=Sum_PI  TsampFilterVariant=InternalTs  TsampNgainVariant=Passthrough  TsampIntegralVariant=Disabled_SignalSpec  ExternalSaturationOutDataTypeStr=Inherit: Same as second input
  Degrees to Radians{,1..9} (10 alike) : simulink_extras/Transformations/Degrees to Radians
  Delay : Delay  DelayLength=1  InitialCondition=0  UseCircularBuffer=on
  Delay1 : Delay  DelayLength=1
  Delay2 : Delay  Commented=on  DelayLength=1
  Delay3 : Delay  Commented=on  DelayLength=1
  Derivative : Derivative
  Derivative1 : Derivative
  Distance from UAV to target and Target coordinate in CAM frame : MATLAB Function  TreatAsAtomicUnit=on
  Divide : Product  Inputs=*/
  From Workspace : FromWorkspace  VariableName=UAV_Roll
  From Workspace1 : FromWorkspace  VariableName=UAV_Pitch
  From Workspace10 : FromWorkspace  VariableName=UAV_Lat
  From Workspace11 : FromWorkspace  VariableName=UAV_Alt
  From Workspace12 : FromWorkspace  VariableName=Target_Lat
  From Workspace13 : FromWorkspace  VariableName=Target_Alt
  From Workspace14 : FromWorkspace  VariableName=Target_Lon
  From Workspace15 : FromWorkspace  VariableName=Distance
  From Workspace2 : FromWorkspace  VariableName=UAV_Yaw
  From Workspace3 : FromWorkspace  VariableName=UAV_Vx
  From Workspace4 : FromWorkspace  VariableName=UAV_Vy
  From Workspace5 : FromWorkspace  VariableName=UAV_Vz
  From Workspace6 : FromWorkspace  VariableName=UAV_p
  From Workspace7 : FromWorkspace  VariableName=UAV_q
  From Workspace8 : FromWorkspace  VariableName=UAV_r
  From Workspace9 : FromWorkspace  VariableName=UAV_Lon
  From22 : From  Commented=on  GotoTag=Ae
  From29 : From  Commented=on  GotoTag=Bk
  Gain1 : Gain  Gain=EL.RotaMoment
  Gain2 : Gain  Gain=AZ.RotaMoment
  Gain3 : Gain  Gain=AZ.BackEMF
  Gain4 : Gain  Gain=EL.BackEMF
  Gain5 : Gain  Gain=EL.RotaMoment
  Gain6 : Gain  Gain=AZ.RotaMoment
  Gain7 : Gain  Gain=AZ.BackEMF
  Gain8 : Gain  Gain=EL.BackEMF
  Gimbal : MATLAB Function  TreatAsAtomicUnit=on
  Goto34 : Goto  Commented=on  GotoTag=TfAz
  Goto35 : Goto  Commented=on  GotoTag=TfEl
  Integrator{,1..3} (4 alike) : Integrator
  Integrator4 : Integrator  Commented=on
  Integrator5 : Integrator  Commented=on
  Kinematic : MATLAB Function  TreatAsAtomicUnit=on
  Longitudinal Velocity of Camera : MATLAB Function  TreatAsAtomicUnit=on
  MATLAB Function : MATLAB Function  Commented=on  TreatAsAtomicUnit=on
  MATLAB Function1 : MATLAB Function  Commented=on  TreatAsAtomicUnit=on
  Mux{,1..3} (4 alike) : Mux  Inputs=2
  Mux4 : Mux  Inputs=3
  Mux5 : Mux  Inputs=3
  Product : Product
  Reshape : Reshape  OutputDimensionality=Column vector (2-D)
  Reshape1 : Reshape  OutputDimensionality=Column vector (2-D)
  Scope{,1..4} (5 alike) : Scope
  Sum{,1..13} (14 alike) : Sum  Inputs=|+-
  Switch : Switch  Criteria=u2 > Threshold  Threshold=5000
  Switch1 : Switch  Criteria=u2 > Threshold  Threshold=5000
  To Workspace : ToWorkspace  VariableName=etaCmd  SaveFormat=Timeseries  SampleTime=-1
  To Workspace1 : ToWorkspace  VariableName=eta  SaveFormat=Timeseries  SampleTime=-1
  To Workspace2 : ToWorkspace  VariableName=epsilonCmd  SaveFormat=Timeseries  SampleTime=-1
  To Workspace3 : ToWorkspace  VariableName=epsilon  SaveFormat=Timeseries  SampleTime=-1
  To Workspace4 : ToWorkspace  VariableName=CEL  SaveFormat=Timeseries  SampleTime=-1
  To Workspace5 : ToWorkspace  VariableName=CELcmd  SaveFormat=Timeseries  SampleTime=-1
  To Workspace6 : ToWorkspace  VariableName=EL  SaveFormat=Timeseries  SampleTime=-1
  To Workspace7 : ToWorkspace  VariableName=ELcmd  SaveFormat=Timeseries  SampleTime=-1
  To Workspace8 : ToWorkspace  VariableName=d  SaveFormat=Timeseries  SampleTime=-1
  Transfer Fcn : TransferFcn  Denominator=[AZ.L AZ.R]
  Transfer Fcn1 : TransferFcn  Denominator=[EL.L EL.R]
  Transfer Fcn2 : TransferFcn  Denominator=[AZ.L AZ.R]
  Transfer Fcn3 : TransferFcn  Denominator=[EL.L EL.R]
  wires:
  Angle controller/1 -> Sum2/1  "omega_ref"
  Sum/1 -> Current controller/1
  Sum2/1 -> Angular velocity controller/1
  Angular velocity controller/1 -> Sum/1  "Iref"
  Current controller/1 -> Sum1/1  "u"
  Gain3/1 -> Sum1/2  "uemf"
  Gain2/1 -> [T_AZ1]  "moment"
  Transfer Fcn/1 -> Sum/2, Gain2/1  "I"
  Sum1/1 -> Transfer Fcn/1
  Sum3/1 -> Current controller1/1
  Angle controller1/1 -> Sum5/1  "omega_ref"
  Angular velocity controller1/1 -> Sum3/1  "Iref"
  Sum5/1 -> Angular velocity controller1/1
  Gain1/1 -> [T_EL1]  "moment"
  Gain4/1 -> Sum4/2  "uemf"
  Current controller1/1 -> Sum4/1  "u"
  Transfer Fcn1/1 -> Sum3/2, Gain1/1  "I"
  Sum4/1 -> Transfer Fcn1/1
  Switch/1 -> Gimbal/1(T_AZ)
  [Ad] -> Gimbal/7(omegaAd)
  [Bk] -> Gimbal/11(omegaBk)
  [Be] -> Gimbal/10(omegaBe)
  [Ar] -> Gimbal/5(omegaAr)
  [Bn] -> Gimbal/8(omegaBn), Derivative1/1
  Derivative/1 -> Gimbal/15(epsilon_dot)
  [r] -> Kinematic/7(yaw)
  Kinematic/6(epsilon_dot) -> Integrator1/1
  Derivative1/1 -> Gimbal/9(omegaBn_dot)
  [Ae] -> Kinematic/4(omegaAe)
  Integrator2/1 -> [Ae]
  Integrator3/1 -> [Bk]
  [p] -> Kinematic/5(roll)
  [q] -> Kinematic/6(pitch)
  [Bk] -> Kinematic/2(omegaBk)
  Gimbal/2(omegaBk_dot) -> Integrator3/1
  Kinematic/2(omegaBe) -> [Be]
  Integrator1/1 -> [epsilon]
  Kinematic/1(omegaBn) -> [Bn]
  [eta] -> Kinematic/1(eta)
  [epsilon] -> Kinematic/3(epsilon)
  Integrator/1 -> [eta]
  Gimbal/1(omegaAe_dot) -> Integrator2/1
  Kinematic/3(omegaAr) -> [Ar]
  Kinematic/5(eta_dot) -> Integrator/1
  [Ae] -> Gimbal/6(omegaAe)
  Kinematic/4(omegaAd) -> [Ad]
  Switch1/1 -> Gimbal/2(T_EL)
  [Bk] -> Sum2/2, Gain3/1
  [Ae] -> Sum5/2, Gain4/1
  Current controller3/1 -> Sum10/1  "u"
  Gain8/1 -> Sum10/2  "uemf"
  Angular velocity controller3/1 -> Sum9/1  "Iref"
  Gain5/1 -> [T_EL2]  "moment"
  Sum11/1 -> Angular velocity controller3/1
  [omegaELcmd] -> Sum11/1  "omega_ref"
  [Bk] -> Gain7/1
  Sum9/1 -> Current controller3/1
  [Ae] -> Sum11/2, Gain8/1
  Sum6/1 -> Current controller2/1
  [omegaCELcmd] -> Sum8/1  "omega_ref"
  Gain7/1 -> Sum7/2  "uemf"
  Sum10/1 -> Transfer Fcn3/1
  Sum8/1 -> Angular velocity controller2/1
  Gain6/1 -> [T_AZ2]  "moment"
  Current controller2/1 -> Sum7/1  "u"
  Transfer Fcn3/1 -> Sum9/2, Gain5/1  "I"
  Transfer Fcn2/1 -> Sum6/2, Gain6/1  "I"
  Sum7/1 -> Transfer Fcn2/1
  From Workspace4/1 -> [Vy]
  From Workspace11/1 -> [UavAlt]
  From Workspace2/1 -> Degrees to Radians1/1
  From Workspace1/1 -> Degrees to Radians2/1
  From Workspace3/1 -> [Vx]
  From Workspace5/1 -> [Vz]
  Degrees to Radians1/1 -> [Yaw]
  Degrees to Radians2/1 -> [Pitch]
  From Workspace13/1 -> [TaAlt]
  From Workspace/1 -> Degrees to Radians/1
  Degrees to Radians/1 -> [Roll]
  [target_CAMbody] -> Azimuth and Elevator Command/3(target_CAMbody)
  [r] -> Longitudinal Velocity of Camera/6(r)
  Distance from UAV to target and Target coordinate in CAM frame/2(target_CAMbody) -> [target_CAMbody]
  [Vx] -> Longitudinal Velocity of Camera/1(Vx)
  Azimuth and Elevator Command/1(psi_AZ_cmd) -> [psi_Az_cmd]
  [q] -> Longitudinal Velocity of Camera/5(q)
  [Vy] -> Longitudinal Velocity of Camera/2(Vy)
  Azimuth and Elevator Command/2(theta_EL_cmd) -> [theta_EL_cmd]
  Longitudinal Velocity of Camera/1(lon_Vel_Cam) -> [lonVelCam]
  [Vz] -> Longitudinal Velocity of Camera/3(Vz)
  [lonVelCam] -> Azimuth and Elevator Command/4(lon_Vel_CAM)
  [UavLo] -> Distance from UAV to target and Target coordinate in CAM frame/2(UAV_Lon)
  [Pitch] -> Distance from UAV to target and Target coordinate in CAM frame/8(pitch)
  [UavAlt] -> Distance from UAV to target and Target coordinate in CAM frame/3(UAV_Alt)
  [TaLon] -> Distance from UAV to target and Target coordinate in CAM frame/5(Target_Lon)
  [eta] -> Distance from UAV to target and Target coordinate in CAM frame/10(psi_AZ)
  [epsilon] -> Distance from UAV to target and Target coordinate in CAM frame/11(theta_EL)
  [Yaw] -> Distance from UAV to target and Target coordinate in CAM frame/9(yaw)
  [p] -> Longitudinal Velocity of Camera/4(p)
  [d] -> Azimuth and Elevator Command/1(distance)
  [UavLat] -> Distance from UAV to target and Target coordinate in CAM frame/1(UAV_Lat)
  [TaAlt] -> Distance from UAV to target and Target coordinate in CAM frame/6(Target_Alt)
  [TaLat] -> Distance from UAV to target and Target coordinate in CAM frame/4(Target_Lat)
  [Roll] -> Distance from UAV to target and Target coordinate in CAM frame/7(roll)
  [psi_Az_cmd] -> Sum12/1
  Sum12/1 -> Angle controller/1
  [theta_EL_cmd] -> Sum13/1
  Sum13/1 -> Angle controller1/1
  [eta] -> Sum12/2
  [epsilon] -> Sum13/2
  [d] -> Switch1/2, Switch/2
  [T_AZ1] -> Switch/1
  [T_AZ2] -> Switch/3
  [T_EL1] -> Switch1/1
  [T_EL2] -> Switch1/3
  [theta_EL_cmd] -> To Workspace2/1, Mux1/1
  [psi_Az_cmd] -> To Workspace/1, Mux/1
  Mux/1 -> Scope/1
  [eta] -> To Workspace1/1, Mux/2
  [epsilon] -> To Workspace3/1, Mux1/2
  Mux1/1 -> Scope1/1
  Mux2/1 -> Scope2/1
  [Ad] -> To Workspace4/1, Mux2/2
  Mux3/1 -> Scope3/1
  [omegaCELcmd] -> To Workspace5/1, Mux2/1
  [omegaELcmd] -> To Workspace7/1, Mux3/1
  [Ae] -> To Workspace6/1, Mux3/2
  [d] -> To Workspace8/1, Scope4/1
  Constant/1 -> Azimuth and Elevator Command/5(Optics_res_width)
  Constant1/1 -> Azimuth and Elevator Command/6(Optics_FOV_rad)
  Mux4/1 -> Reshape/1
  Mux5/1 -> Reshape1/1
  Reshape/1 -> Gimbal/12(AZ)
  Reshape1/1 -> Gimbal/13(EL)
  Constant7/1 -> Mux5/3
  Constant6/1 -> Mux5/2
  Constant5/1 -> Mux5/1
  Constant4/1 -> Mux4/3
  Constant3/1 -> Mux4/2
  Constant2/1 -> Mux4/1
  From Workspace6/1 -> Degrees to Radians3/1
  Degrees to Radians3/1 -> [p]
  From Workspace7/1 -> Degrees to Radians4/1
  Degrees to Radians4/1 -> [q]
  From Workspace8/1 -> Degrees to Radians5/1
  Degrees to Radians5/1 -> [r]
  Degrees to Radians7/1 -> [UavLo]
  From Workspace9/1 -> Degrees to Radians7/1
  Degrees to Radians6/1 -> [UavLat]
  From Workspace10/1 -> Degrees to Radians6/1
  Degrees to Radians9/1 -> [TaLon]
  From Workspace14/1 -> Degrees to Radians9/1
  From Workspace12/1 -> Degrees to Radians8/1
  Degrees to Radians8/1 -> [TaLat]
  From Workspace15/1 -> [d]
  [epsilon] -> Delay/1
  Delay/1 -> Gimbal/14(epsilon), Derivative/1
  [Ar] -> Delay1/1
  Delay1/1 -> Azimuth and Elevator Command/2(omegaEx)
  [Ad] -> Sum8/2
  Azimuth and Elevator Command/3(omega_CEL_cmd) -> [omegaCELcmd]
  Azimuth and Elevator Command/4(omega_EL_cmd) -> [omegaELcmd]
  [epsilon] -> Cos/1
  Constant8/1 -> Divide/1
  Cos/1 -> Divide/2
  Angular velocity controller2/1 -> Product/1  "Iref"
  Product/1 -> Sum6/1
  Divide/1 -> Product/2
  MATLAB Function/2(z_dot) -> Integrator4/1
  Integrator4/1 -> MATLAB Function/4(z)
  MATLAB Function1/2(z_dot) -> Integrator5/1
  Integrator5/1 -> MATLAB Function1/4(z)
  MATLAB Function/1(TfAz) -> Goto34/1
  MATLAB Function1/1(TfEl) -> Goto35/1
  Constant9/1 -> MATLAB Function/1(sigma2)
  Constant11/1 -> MATLAB Function1/1(sigma2)
  From29/1 -> Delay2/1
  Delay2/1 -> MATLAB Function/3(omega)
  Constant10/1 -> MATLAB Function/2(AZomega_s)
  From22/1 -> Delay3/1
  Delay3/1 -> MATLAB Function1/3(omega)
  Constant12/1 -> MATLAB Function1/2(ELomega_s)
  [eta] -> Longitudinal Velocity of Camera/7(psi_AZ)
  [epsilon] -> Longitudinal Velocity of Camera/8(theta_EL)
  Constant13/1 -> Gimbal/4(TfEl), Gimbal/3(TfAz)

== matlab function LOS_Tracking/MATLAB Function ==
  data: sigma2 input; TfAz output; AZomega_s input; omega input; z input; z_dot output
function [TfAz, z_dot] = LuGre_Friction(sigma2, AZomega_s, omega, z)
%==========================================================================
% LuGre Dynamic Friction Model
%
% Input:
%   omega : Angular velocity (rad/s)
%   z     : Internal LuGre state (Integrator output)
%
% Output:
%   TfAz    : Friction torque (N.m)
%   z_dot : State derivative
%
%==========================================================================

%% Parameters
Fc      = 0.02;      % Coulomb friction torque (N.m)
Fs      = 0.03;      % Static friction torque (N.m)

sigma0  = 1000;      % Bristle stiffness
sigma1  = 10;        % Bristle damping


%% Stribeck Function

g = (Fc + (Fs - Fc)*exp(-(omega/AZomega_s)^2))/sigma0;

%% LuGre State Equation

z_dot = omega - abs(omega)/g*z;

%% Friction Torque

TfAz = 0; %sigma0*z + sigma1*z_dot + sigma2*omega;

end

== matlab function LOS_Tracking/MATLAB Function1 ==
  data: sigma2 input; TfEl output; ELomega_s input; omega input; z input; z_dot output
function [TfEl, z_dot] = LuGre_Friction(sigma2, ELomega_s, omega, z)
%==========================================================================
% LuGre Dynamic Friction Model
%
% Input:
%   omega : Angular velocity (rad/s)
%   z     : Internal LuGre state (Integrator output)
%
% Output:
%   TfAz    : Friction torque (N.m)
%   z_dot : State derivative
%
%==========================================================================

%% Parameters
Fc      = 0.02;      % Coulomb friction torque (N.m)
Fs      = 0.03;      % Static friction torque (N.m)

sigma0  = 1000;      % Bristle stiffness
sigma1  = 10;        % Bristle damping


%% Stribeck Function

g = (Fc + (Fs - Fc)*exp(-(omega/ELomega_s)^2))/sigma0;

%% LuGre State Equation

z_dot = omega - abs(omega)/g*z;

%% Friction Torque

TfEl = 0; %sigma0*z + sigma1*z_dot + sigma2*omega;

end

== matlab function LOS_Tracking/Azimuth and Elevator Command ==
  data: psi_AZ_cmd output; theta_EL_cmd output; distance input; omega_CEL_cmd output; omega_EL_cmd output; omegaEx input; target_CAMbody input; lon_Vel_CAM input; Optics_res_width input; Optics_FOV_rad input
function [psi_AZ_cmd, theta_EL_cmd, omega_CEL_cmd, omega_EL_cmd] = Azimuth_Elevator(distance, omegaEx, target_CAMbody, lon_Vel_CAM, Optics_res_width, Optics_FOV_rad)
    % =====================================================================
    % HÀM TÍNH GÓC ĐƯỜNG NGẮM (LOS) VÀ CHUYỂN ĐỔI TRẠNG THÁI TÁC CHIẾN
    %
    % Đầu vào:
    %   - target_body: Vector 3D [x_b; y_b; z_b] từ hàm tính WGS84 trước đó
    %   - distance: Khoảng cách hiện tại đến mục tiêu (m)
    %
    % Đầu ra:
    %   - psi_AZ_cmd: Lệnh góc quay Azimuth (Radian) cấp cho Gimbal
    %   - theta_EL_cmd: Lệnh góc ngẩng Elevation (Radian) cấp cho Gimbal
    %   - omega_AZ_cmd: vận tốc góc quay Azimuth (Radian/s) cấp cho Gimbal
    %   - omega_EL_cmd: vận tốc góc ngẩng Elevation (Radian/s) cấp cho Gimbal
    % =====================================================================
    %% Khởi tạo
    psi_AZ_cmd = 0;
    theta_EL_cmd = 0;
    omega_CEL_cmd = 0;
    omega_EL_cmd = 0;
    
    alpha = 0.25;
    omega_ROT = omegaEx;  % omegaEx = omegaAr 

    %% Vận tốc dài của camera
    vx_c = lon_Vel_CAM(1);
    vy_c = lon_Vel_CAM(2);
    vz_c = lon_Vel_CAM(3);
    %% Image tracking
    % Tọa độ của Target trong hệ tọa độ Camera
    x_c = target_CAMbody(1);
    y_c = target_CAMbody(2);
    z_c = target_CAMbody(3);

    % Tính toán tiêu cự của camera
    lambda = Optics_res_width / (2 * tan(Optics_FOV_rad / 2));

    % Mô hình lỗ kim (Pinhole)
    u = lambda * (x_c / z_c);
    w = lambda * (y_c / z_c);

    % Tính mẫu số chung 
    mau_so_chung = lambda^2 + u^2 + w^2;
    mau_so_z = z_c * mau_so_chung;

    %% 1. Phương trình cho omega_EL_ref
    term1_EL = (alpha * w * lambda) / mau_so_chung;
    term2_EL = (omega_ROT * u) / lambda;
    tu_so_3_EL = (lambda^2 * vy_c) - (lambda * w * vz_c) - (u * w * vx_c) + (u^2 * vy_c);
    term3_EL = tu_so_3_EL / mau_so_z;

    omega_EL_ref = term1_EL - term2_EL - term3_EL;

    %% 2. Phương trình cho omega_CEL_ref
    term1_CEL = -(alpha * u * lambda) / mau_so_chung;
    term2_CEL = (omega_ROT * w) / lambda;
    tu_so_3_CEL = (lambda^2 * vx_c) - (lambda * u * vz_c) - (w * u * vy_c) + (w^2 * vx_c);
    term3_CEL = tu_so_3_CEL / mau_so_z;

    omega_CEL_ref = term1_CEL - term2_CEL + term3_CEL;
    
    %% Logic chuyển trạng thái
    if distance > 5000
        % GIAI ĐOẠN 1: Hành trình (Distance > 5km)
        % Khóa cứng Gimbal ở 0 độ so với trục dọc máy bay
        psi_AZ_cmd = 0;             % eta = 0
        theta_EL_cmd = 0;           % epsilon = 0
    else
        % GIAI ĐOẠN 2: Homing (Distance <= 5km)
        % Mở khóa, bắt đầu bám theo góc LOS
        omega_CEL_cmd = omega_CEL_ref;
        omega_EL_cmd = omega_EL_ref;
    end

end

== matlab function LOS_Tracking/Distance from UAV to target and Target coordinate in CAM frame ==
  data: UAV_Lat input; distance output; UAV_Lon input; UAV_Alt input; Target_Lat input; Target_Lon input; Target_Alt input; roll input; pitch input; yaw input; target_CAMbody output; psi_AZ input; theta_EL input
function [distance, target_CAMbody] = Distance(UAV_Lat, UAV_Lon, UAV_Alt, Target_Lat, Target_Lon, Target_Alt, roll, pitch, yaw, psi_AZ, theta_EL)
    % =====================================================================
    % HÀM TÍNH TOÁN KHOẢNG CÁCH VÀ TỌA ĐỘ MỤC TIÊU (CHUẨN WGS84)
    % 
    % Đầu vào:
    %   - UAV_Lat, UAV_Lon, UAV_Alt: Tọa độ GPS của máy bay (Radian, Mét)
    %   - Target_Lat, Target_Lon, Target_Alt: Tọa độ GPS của mục tiêu (Radian, Mét)
    %   - roll, pitch, yaw: Tư thế góc Euler của máy bay (Radian)
    % 
    % Đầu ra:
    %   - distance: Khoảng cách đường thẳng từ UAV đến mục tiêu (Mét)
    %   - target_UAVbody: Vector tọa độ 3D của mục tiêu trong hệ quy chiếu 
    %                  thân UAV [x_b; y_b; z_b]
    %   - target_CAMbody: Vector tọa độ 3D của mục tiêu trong hệ quy chiếu 
    %                  Camera [x_c; y_c; z_c]
    % =====================================================================

    %% 1. HẰNG SỐ TRÁI ĐẤT (HỆ WGS84)
    R0 = 6378137.0; % Bán kính xích đạo (m)
    e = 0.0818191908425; % Độ lệch tâm

    % Tính bán kính cong hình đứng chuẩn tại vị trí UAV và Target
    R_E_base = R0 / sqrt(1 - (e * sin(UAV_Lat))^2) ; 
    R_E_target = R0 / sqrt(1 - (e * sin(Target_Lat))^2) ; 

    %% 2. CHUYỂN ĐỔI SANG HỆ TỌA ĐỘ ĐỀ CÁC (ECEF)
    % ECEF UAV (Base)
    x_base_ECEF = (R_E_base + UAV_Alt) * cos(UAV_Lat) * cos(UAV_Lon);
    y_base_ECEF = (R_E_base + UAV_Alt) * cos(UAV_Lat) * sin(UAV_Lon);
    z_base_ECEF = ( (1 - e^2) * R_E_base + UAV_Alt ) * sin(UAV_Lat);
    
    % ECEF Mục tiêu (Target)
    x_target_ECEF = (R_E_target + Target_Alt) * cos(Target_Lat) * cos(Target_Lon);
    y_target_ECEF = (R_E_target + Target_Alt) * cos(Target_Lat) * sin(Target_Lon);
    z_target_ECEF = ( (1 - e^2) * R_E_target + Target_Alt ) * sin(Target_Lat);
    
    base_ECEF = [x_base_ECEF; y_base_ECEF; z_base_ECEF];
    target_ECEF = [x_target_ECEF; y_target_ECEF; z_target_ECEF];
    
    % Vector khoảng cách trong hệ ECEF
    base_to_target_ECEF = target_ECEF - base_ECEF;
    
    % XUẤT KẾT QUẢ 1: KHOẢNG CÁCH EUCLID
    distance = sqrt(base_to_target_ECEF(1,1)^2 + base_to_target_ECEF(2,1)^2 + base_to_target_ECEF(3,1)^2);

    %% 3. CHUYỂN ĐỔI ECEF -> HỆ TỌA ĐỘ PHẲNG ĐỊA PHƯƠNG (LNF / NED)
    % Sử dụng tọa độ gốc là UAV
    ECEF_to_LNF_matrix = [
        -sin(UAV_Lat)*cos(UAV_Lon), -sin(UAV_Lat)*sin(UAV_Lon),  cos(UAV_Lat);
        -sin(UAV_Lon),              cos(UAV_Lon),              0;
        -cos(UAV_Lat)*cos(UAV_Lon), -cos(UAV_Lat)*sin(UAV_Lon), -sin(UAV_Lat)
    ];
    
    base_to_target_LNF = ECEF_to_LNF_matrix * base_to_target_ECEF;

    %% 4. CHUYỂN ĐỔI LNF -> HỆ TỌA ĐỘ THÂN (BODY FRAME)
    % Xoay theo các góc Euler của UAV
    LNF_to_body_matrix = [
        cos(pitch)*cos(yaw), ...
        cos(pitch)*sin(yaw), ...
        -sin(pitch);
        
        sin(roll)*sin(pitch)*cos(yaw) - cos(roll)*sin(yaw), ...
        sin(roll)*sin(pitch)*sin(yaw) + cos(roll)*cos(yaw), ...
        sin(roll)*cos(pitch);
        
        cos(roll)*sin(pitch)*cos(yaw) + sin(roll)*sin(yaw), ...
        cos(roll)*sin(pitch)*sin(yaw) - sin(roll)*cos(yaw), ...
        cos(roll)*cos(pitch)
    ];
    
    % XUẤT KẾT QUẢ 2: VECTOR VỊ TRÍ MỤC TIÊU SO VỚI THÂN UAV
    target_UAVbody = LNF_to_body_matrix * base_to_target_LNF;

    %% 5. CHUYỂN ĐỔI BODY FRAME -> HỆ TỌA ĐỘ CAMERA (CAMERA FRAME)
    % Khung Gimbal AZ quay quanh trục Z của thân UAV một góc theta_AZ
    Body_to_AZ_matrix = [
        cos(psi_AZ),  sin(psi_AZ), 0;
       -sin(psi_AZ),  cos(psi_AZ), 0;
        0,              0,             1
    ];

    % Khung Gimbal EL (gắn Camera) quay quanh trục Y của khung AZ một góc theta_EL
    AZ_to_Camera_matrix = [
        cos(theta_EL), 0, -sin(theta_EL);
        0,             1,  0;
        sin(theta_EL), 0,  cos(theta_EL)
    ];

    % XUẤT KẾT QUẢ 2: VECTOR VỊ TRÍ MỤC TIÊU TRONG HỆ CAMERA
    % Vector này đã hoàn toàn tách biệt khỏi các nhiễu động của thân UAV và góc quay Gimbal
    target_CAMbody = AZ_to_Camera_matrix * Body_to_AZ_matrix * target_UAVbody;

end
